simulink model "Boost_28V_simple"  (R2021b)
settings: Solver=FixedStepDiscrete  StartTime=0.0  StopTime=0.02  FixedStep=1/(477600*128)  RelTol=1e-3
libraries: spsSeriesRLCBranchLib x3, simulink x2, spsDiodeLib x1, spsGroundLib x1, spsCurrentMeasurementLib x1, spsIdealSwitchLib x1, spsDCVoltageSourceLib x1, spsVoltageMeasurementLib x1, spspowerguiLib x1
settings Model: Creator=wu330  LastModifiedBy=wu330
settings DataIOCC: SaveOutput=off  SaveTime=off

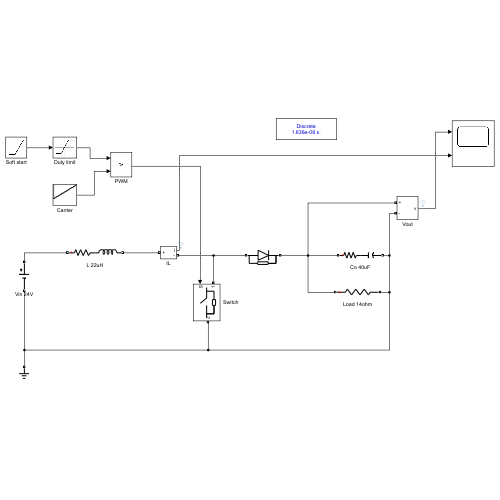
[thumbnail: Simulink's stored preview of the top-level diagram]
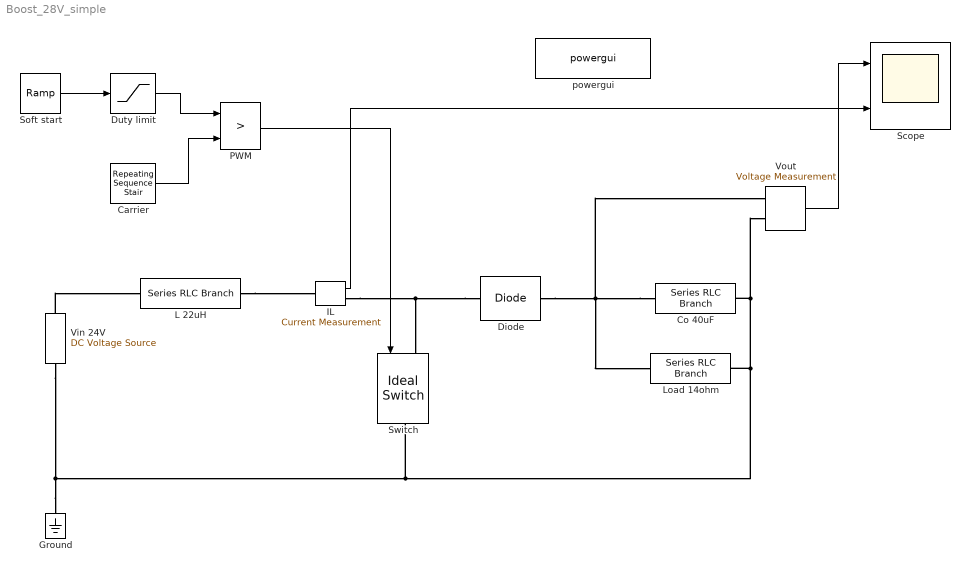
== system Boost_28V_simple ==
  Carrier : simulink/Sources/Repeating Sequence Stair  OutValues=((0:127)+0.5)/128  tsamp=1/(477600*128)  OutMin=[]  OutMax=[]  OutDataTypeStr=double  OutputDataTypeScalingMode=double  OutDataType=fixdt(0,8)  ConRadixGroup=Best Precision: Vector-wise  OutScaling=2^-12
  Co 40uF : spsSeriesRLCBranchLib/Series RLC Branch  LConnTagsString=__new0  RConnTagsString=__new0  BranchType=RC  Resistance=0.01  Inductance=1e-3  SetiL0=off  InitialCurrent=0  Capacitance=40e-6  Setx0=on  InitialVoltage=(24-0.5)/(1+(0.074+0.001)/14)  Measurements=None
  Diode : spsDiodeLib/Diode  Ron=0.001  Lon=0  Vf=0.5  IC=0  UseSnubber=0  Rs=500  Cs=250e-9  Measurements=off
  Duty limit : Saturate  UpperLimit=21/128  LowerLimit=0
  Ground : spsGroundLib/Ground  LConnTagsString=a
  IL : spsCurrentMeasurementLib/Current Measurement  PhasorSimulation=off  OutputType=Complex  PSBequivalent=0
  L 22uH : spsSeriesRLCBranchLib/Series RLC Branch  LConnTagsString=__new0  RConnTagsString=__new0  BranchType=RL  Resistance=0.074  Inductance=22e-6  SetiL0=on  InitialCurrent=(24-0.5)/(14+0.074+0.001)  Capacitance=1e-6  Setx0=off  InitialVoltage=0  Measurements=None
  Load 14ohm : spsSeriesRLCBranchLib/Series RLC Branch  LConnTagsString=__new0  RConnTagsString=__new0  BranchType=R  Resistance=14  Inductance=1e-3  SetiL0=off  InitialCurrent=0  Capacitance=1e-6  Setx0=off  InitialVoltage=0  Measurements=None
  PWM : RelationalOperator  Operator=>  OutDataTypeStr=boolean  RndMeth=Simplest
  Scope : Scope  NumInputPorts=2
  Soft start : simulink/Sources/Ramp  slope=(21/128)/0.005  start=0.003  InitialOutput=0
  Switch : spsIdealSwitchLib/Ideal Switch  Ron=0.06  Lon=0  IC=0  Rs=1e6  Cs=inf  Measurements=off
  Vin 24V : spsDCVoltageSourceLib/DC Voltage Source  Amplitude=24  Measurements=None
  Vout : spsVoltageMeasurementLib/Voltage Measurement  PhasorSimulation=off  OutputType=Complex  PSBequivalent=0
  powergui : spspowerguiLib/powergui  Priority=1  SimulationMode=Discrete  SampleTime=1/(477600*128)  frequency=60  Iterations=50  frequencyindice=60  Pbase=100e6  ErrMax=1e-4  UnitsV=kV  UnitsW=MW  buscounter=0  FunctionMessages=off  echomessages=off  EnableUseOfTLC=off  CurrentSourceSwitches=off  DisableSnubberDevices=off  DisableRonSwitches=off  DisableVfSwitches=off  DisplayEquations=off  AutomaticDiscreteSolvers=off  SolverType=Tustin/Backward Euler (TBE)  Interpol=off  ExternalGateDelay=off  methode=off  Ts=100  x0status=blocks  SPID=on  SwTol=0  HookPort=off  NonlinearTolerance=1e-4  nMaxIteration=100  ContinueOnMaxIteration=off  RestoreLinks=warning  ResistiveCurrentMeasurement=off  Frange=[0:2:500]  Ylog=off  Xlog=on  ShowGrid=off  save=off  variable=ZData  structure=0  ZoomFFT=off  StartTime=0.0  cycles=1  DisplayStyle=1  fundamental=60  FreqAxis=off  MaxFrequency=1000  frequencyindicesteady=1  RmsSteady=1  display=off
  wires:
  Soft start/1 -> Duty limit/1
  Duty limit/1 -> PWM/1
  Carrier/1 -> PWM/2
  PWM/1 -> Switch/1
  Vout/1 -> Scope/1
  IL/1 -> Scope/2
  connections:
  Vin 24V/RConn1 -- L 22uH/LConn1
  L 22uH/RConn1 -- IL/LConn1
  Diode/LConn1 -- IL/RConn1 -- Switch/LConn1
  Co 40uF/LConn1 -- Vout/LConn1 -- Diode/RConn1 -- Load 14ohm/LConn1
  Ground/LConn1 -- Vin 24V/LConn1 -- Switch/RConn1 -- Vout/LConn2 -- Co 40uF/RConn1 -- Load 14ohm/RConn1
